simulink model "grad_V2"  (R2024a)
settings: Solver=FixedStepAuto  StartTime=0.0  StopTime=inf  RelTol=1e-3  EnableMultiTasking=on
InitFcn:
  | Ts=0.01;
  | RE=165; % count per cm
  | L=30; %cm
undefined symbols (not defined in the file or in its folder): DiscIntNeverNeededParam
libraries: arduinolib x6, arduinosensorlib x2, slpidlib x1, arduinowifilib x1
settings Model: ExtModeTrigDuration=2  Creator=andrew  LastModifiedBy=andrew
settings SolverCC: AutoInsertRateTranBlk=on
settings OptimizationCC: EnhancedBackFolding=on  PassReuseOutputArgsAs=Individual arguments  ZeroExternalMemoryAtStartup=off  ZeroInternalMemoryAtStartup=off  MaxStackSize=64  OptimizeBlockOrder=speed  DifferentSizesBufferReuse=on  OptimizationCustomize=off  EfficientTunableParamExpr=on
settings DebuggingCC: MultiTaskDSMMsg=none  ParameterTunabilityLossMsg=error
settings HardwareCC: ProdBitPerPointer=32  ProdBitPerSizeT=32  ProdBitPerPtrDiffT=32  ProdLargestAtomicInteger=Long  ProdLargestAtomicFloat=Double  ProdWordSize=32  ProdHWDeviceType=ARM Compatible->ARM Cortex
settings SFSimCC: MATLABDynamicMemAlloc=off
settings RTWCC: Description=Embedded Coder  SystemTargetFile=ert.tlc  HardwareBoard=ESP32-WROOM(Arduino Compatible)  TLCOptions="-aInlineSetEventsForThisBaseRateFcn=TLC_FALSE -aSuppressMultiTaskScheduler=TLC_FALSE  -aRateBasedStepFcn=0"  TemplateMakefile=ert_default_tmf  Toolchain=ESP32  BuildConfiguration=Faster Runs
settings CodeAppCC: ForceParamTrailComments=on  IgnoreCustomStorageClasses=off  OperatorAnnotations=on  SimulinkDataObjDesc=on  SFDataObjDesc=on  InsertBlockDesc=on
settings ERTTargetCC: SupportContinuousTime=on  SupportVariableSizeSignals=on  ExtModeTransport=3  ExtModeStaticAlloc=on  ExtModeAutomaticAllocSize=off  ExtModeStaticAllocSize=65536  ExtModeMexFile=ext_xcp  ExtModeIntrfLevel=Level2 - Open

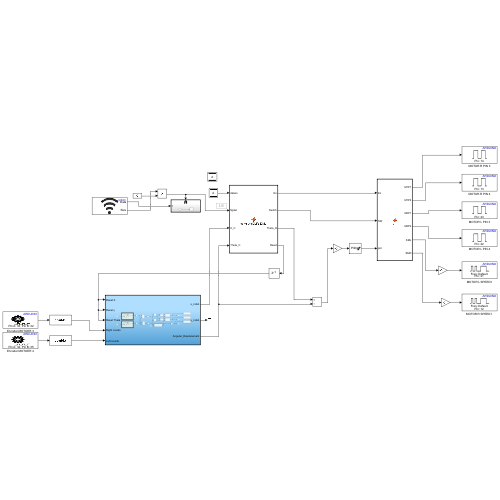
[thumbnail: Simulink's stored preview of the top-level diagram]
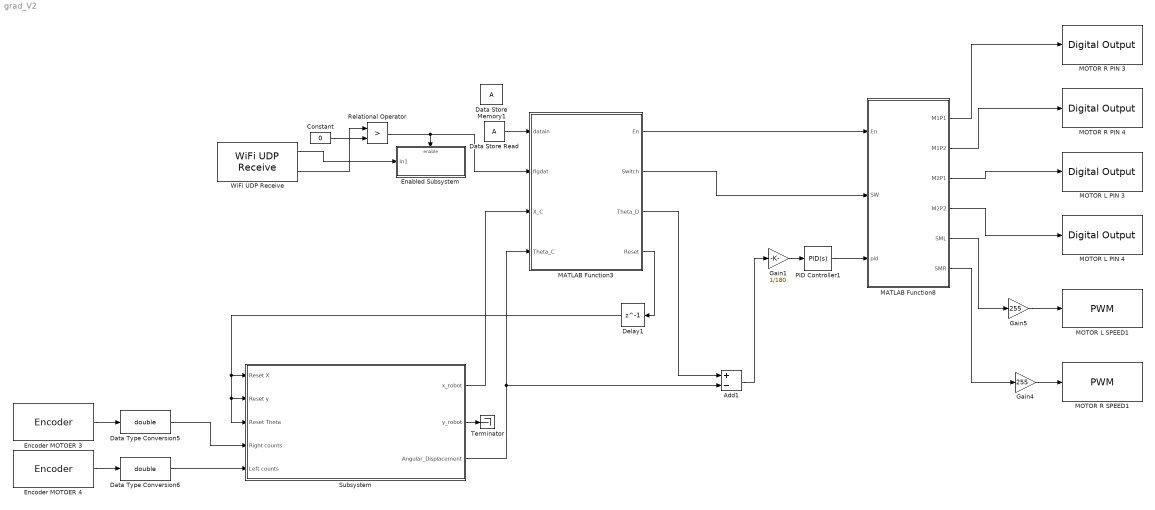
== system grad_V2 ==
  Add1 : Sum  Inputs=+-
  Constant : Constant  Value=0  OutDataTypeStr=uint16
  Data Store Memory1 : DataStoreMemory  WriteAfterWriteMsg=warning  ShowAdditionalParam=off  OutDataTypeStr=uint8  Dimensions=[20 1]
  Data Store Read : DataStoreRead  IndexOptions=Index vector (dialog)  Indices=1  OutputSizes=1
  Data Type Conversion5 : DataTypeConversion  OutDataTypeStr=double  SaturateOnIntegerOverflow=off  RndMeth=Floor
  Data Type Conversion6 : DataTypeConversion  OutDataTypeStr=double  SaturateOnIntegerOverflow=off  RndMeth=Floor
  Delay1 : Delay  DelayLength=1
  Enabled Subsystem : Subsystem  TreatAsAtomicUnit=on
  Encoder MOTOER 3 : arduinosensorlib/Encoder  InputA=33  InputB=32  Mode=No reset  SampleTime=-1
  Encoder MOTOER 4 : arduinosensorlib/Encoder  InputA=34  InputB=35  Mode=No reset  SampleTime=-1
  Gain1 : Gain  Gain=1/180
  Gain4 : Gain  Gain=255
  Gain5 : Gain  Gain=255
  MATLAB Function3 : MATLAB Function  TreatAsAtomicUnit=on
  MATLAB Function8 : MATLAB Function  TreatAsAtomicUnit=on
  MOTOR L PIN 3 : arduinolib/Digital Output  pinNumber=23  Direction=output  blockPlatform=arduino
  MOTOR L PIN 4 : arduinolib/Digital Output  pinNumber=22  Direction=output  blockPlatform=arduino
  MOTOR L SPEED1 : arduinolib/PWM  pinNumber=21  frequencyType=Default  desiredFrequency=490.2  achievableFrequency=490.2
  MOTOR R PIN 3 : arduinolib/Digital Output  pinNumber=14  Direction=output  blockPlatform=arduino
  MOTOR R PIN 4 : arduinolib/Digital Output  pinNumber=13  Direction=output  blockPlatform=arduino
  "MOTOR R SPEED1 " : arduinolib/PWM  pinNumber=12  frequencyType=Default  desiredFrequency=490.2  achievableFrequency=490.2
  PID Controller1 : slpidlib/PID Controller  Controller=PID  Form=Parallel  TimeDomain=Continuous-time  UseExternalTs=off  SampleTime=-1  IntegratorMethod=Forward Euler  FilterMethod=Forward Euler  ControllerParametersSource=internal  P=50  I=5  UseKiTs=off  D=0  UseExternalDerivativeSource=off  N=100  UseFilter=on  TunerSelectOption=Transfer Function Based (PID Tuner App)  InitialConditionSource=internal  InitialConditionForIntegrator=0  InitialConditionForFilter=0  DifferentiatorICPrevScaledInput=0  ExternalReset=none  TrackingMode=off  Kt=1  LimitOutput=on  SatLimitsSource=internal  UpperSaturationLimit=1  LowerSaturationLimit=-1  LinearizeAsGain=on  AntiWindupMode=none  Kb=1  LimitIntegrator=off  UpperIntegratorSaturationLimit=inf  LowerIntegratorSaturationLimit=-inf  POutMin=[]  POutMax=[]  IOutMin=[]  IOutMax=[]  DOutMin=[]  DOutMax=[]  NOutMin=[]  NOutMax=[]  SumOutMin=[]  SumOutMax=[]  SaturationOutMin=[]  SaturationOutMax=[]  PParamMin=[]  PParamMax=[]  IParamMin=[]  IParamMax=[]  DParamMin=[]  DParamMax=[]  NParamMin=[]  NParamMax=[]  KbParamMin=[]  KbParamMax=[]  KtParamMin=[]  KtParamMax=[]  KbOutMin=[]  KbOutMax=[]  KtOutMin=[]  KtOutMax=[]  IntegratorOutMin=[]  IntegratorOutMax=[]  FilterOutMin=[]  FilterOutMax=[]  SumI1OutMin=[]  SumI1OutMax=[]  SumI2OutMin=[]  SumI2OutMax=[]  SumI3OutMin=[]  SumI3OutMax=[]  SumI4OutMin=[]  SumI4OutMax=[]  SumDOutMin=[]  SumDOutMax=[]  DifferentiatorOutMin=[]  DifferentiatorOutMax=[]  FilterDiffOutCoefMin=[]  FilterDiffOutCoefMax=[]  ReciprocalOutMin=[]  ReciprocalOutMax=[]  SumDenOutMin=[]  SumDenOutMax=[]  SumNumOutMin=[]  SumNumOutMax=[]  DivideOutMin=[]  DivideOutMax=[]  UdiffTsProdOutMin=[]  UdiffTsProdOutMax=[]  NTsProdOutMin=[]  NTsProdOutMax=[]  UintegralTsProdOutMin=[]  UintegralTsProdOutMax=[]  UngainTsProdOutMin=[]  UngainTsProdOutMax=[]  ClampingZeroOutDataTypeStr=Inherit: Inherit via back propagation  ClampingZeroOutMin=[]  ClampingZeroOutMax=[]  FilterDenConstantOutDataTypeStr=Inherit: Inherit via back propagation  FilterDenConstantOutMin=[]  FilterDenConstantOutMax=[]  PCopyOutDataTypeStr=Inherit: Inherit via back propagation  PCopyOutMin=[]  PCopyOutMax=[]  NCopyOutDataTypeStr=Inherit: Inherit via back propagation  NCopyOutMin=[]  NCopyOutMax=[]  IntegratorContinuousStateAttributes=''  IntegratorStateMustResolveToSignalObject=off  IntegratorRTWStateStorageClass=Auto  FilterContinuousStateAttributes=''  FilterStateMustResolveToSignalObject=off  FilterRTWStateStorageClass=Auto  ParallelPVariant=InternalParameters  IdealPVariant=Disabled  IVariant=InternalParameters  DVariant=InternalParameters  IntegratorVariant=Continuous  SatVariant=Enabled  AWVariant=Passthrough  PCopyVariant=Disabled  TRVariant=Disabled  FdbkBlocksVariant=Forward  IdealPFdbkVariant=Disabled  SatFdbkVariant=Disabled  DerivativeFilterVariant=ContFilter  NVariant=InternalParameters  NCopyVariant=Disabled  FilterICVariant=InternalICsFilter  IntegratorICVariant=InternalICs  ExternalResetVariant=Disabled  TRSumVariant=Passthrough  SumFdbkVariant=Disabled  SumVariant=Sum_PID  TsampFilterVariant=InternalTs  TsampNgainVariant=Passthrough  TsampIntegralVariant=Disabled_SignalSpec  ExternalSaturationOutDataTypeStr=Inherit: Same as second input  DerivativeSourceVariant=ErrorSignal
  Relational Operator : RelationalOperator  Operator=>  OutDataTypeStr=boolean  RndMeth=Simplest  InputSameDT=off
  Subsystem : Subsystem  TreatAsAtomicUnit=on  SystemSampleTime=Ts
  Terminator : Terminator
  WiFi UDP Receive : arduinowifilib/WiFi UDP Receive  localport=50002  DataType=uint8  DataLength=20  SampleTime_=0.1  wifiUDPIndex=0  blockPlatform=ARDUINO  isARMArch=false
  wires:
  Subsystem/3(Angular_Displacement) -> MATLAB Function3/4(Theta_C), Add1/2
  WiFi UDP Receive/1 -> Enabled Subsystem/1(In1)
  MATLAB Function8/4(M2P2) -> MOTOR L PIN 4/1
  MATLAB Function3/4(Reset) -> Delay1/1
  Constant/1 -> Relational Operator/2
  WiFi UDP Receive/2 -> Relational Operator/1
  MATLAB Function8/3(M2P1) -> MOTOR L PIN 3/1
  MATLAB Function8/6(SMR) -> Gain4/1
  Data Store Read/1 -> MATLAB Function3/1(datain)
  MATLAB Function8/1(M1P1) -> MOTOR R PIN 3/1
  Encoder MOTOER 3/1 -> Data Type Conversion5/1
  Gain5/1 -> MOTOR L SPEED1/1
  Relational Operator/1 -> MATLAB Function3/2(flgdat), Enabled Subsystem/Enable
  MATLAB Function8/5(SML) -> Gain5/1
  Encoder MOTOER 4/1 -> Data Type Conversion6/1
  MATLAB Function3/2(Switch) -> MATLAB Function8/2(SW)
  Add1/1 -> Gain1/1
  MATLAB Function3/1(En) -> MATLAB Function8/1(En)
  Subsystem/2(y_robot) -> Terminator/1
  Data Type Conversion5/1 -> Subsystem/4(Right counts)
  Delay1/1 -> Subsystem/3(Reset Theta), Subsystem/2(Reset y), Subsystem/1(Reset X)
  Gain4/1 -> "MOTOR R SPEED1 "/1
  Subsystem/1(x_robot) -> MATLAB Function3/3(X_C)
  Gain1/1 -> PID Controller1/1
  MATLAB Function8/2(M1P2) -> MOTOR R PIN 4/1
  MATLAB Function3/3(Theta_D) -> Add1/1
  PID Controller1/1 -> MATLAB Function8/3(pid)
  Data Type Conversion6/1 -> Subsystem/5(Left counts)

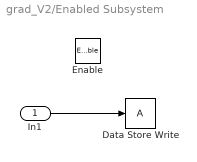
== system grad_V2/Enabled Subsystem ==
  In1 : Inport
  Enable : EnablePort
  Data Store Write : DataStoreWrite  IndexOptions=Index vector (dialog)  Indices=1  OutputSizes=1
  wires:
  In1/1 -> Data Store Write/1

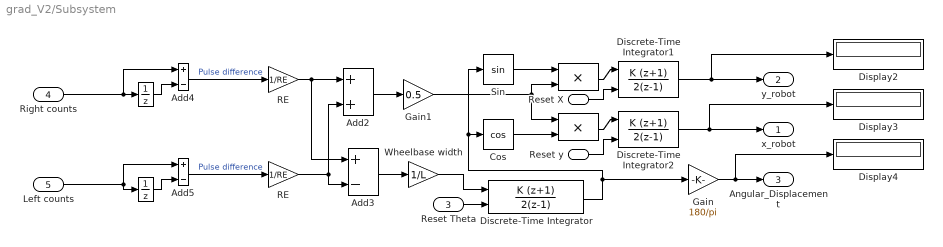
== system grad_V2/Subsystem ==
  Reset X : Inport
  Reset y : Inport  Port=2
  Reset Theta : Inport  Port=3
  Right counts : Inport  Port=4
  Left counts : Inport  Port=5
  " " : Product
  "  " : Product
  "     " : UnitDelay  SampleTime=-1  HasFrameUpgradeWarning=on
  "       " : UnitDelay  SampleTime=-1  HasFrameUpgradeWarning=on
  Add2 : Sum
  Add3 : Sum  Inputs=+-
  Add4 : Sum  Inputs=+-
  Add5 : Sum  Inputs=+-
  Cos : Trigonometry  Operator=cos  ApproximationMethod=CORDIC
  Discrete-Time Integrator : DiscreteIntegrator  IntegratorMethod=Accumulation: Trapezoidal  ExternalReset=level  SampleTime=-1  ICPrevOutput=DiscIntNeverNeededParam  ICPrevScaledInput=DiscIntNeverNeededParam
  Discrete-Time Integrator1 : DiscreteIntegrator  IntegratorMethod=Accumulation: Trapezoidal  ExternalReset=level  SampleTime=-1  ICPrevOutput=DiscIntNeverNeededParam  ICPrevScaledInput=DiscIntNeverNeededParam
  Discrete-Time Integrator2 : DiscreteIntegrator  IntegratorMethod=Accumulation: Trapezoidal  ExternalReset=level  SampleTime=-1  ICPrevOutput=DiscIntNeverNeededParam  ICPrevScaledInput=DiscIntNeverNeededParam
  Display2 : Display
  Display3 : Display
  Display4 : Display
  Gain : Gain  Gain=180/pi
  Gain1 : Gain  Gain=0.5
  "RE  " : Gain  Gain=1/RE
  "RE    " : Gain  Gain=1/RE
  Sin : Trigonometry  ApproximationMethod=CORDIC
  "Wheelbase width " : Gain  Gain=1/L
  x_robot : Outport  VectorParamsAs1DForOutWhenUnconnected=off
  y_robot : Outport  Port=2  VectorParamsAs1DForOutWhenUnconnected=off
  Angular_Displacement : Outport  Port=3  VectorParamsAs1DForOutWhenUnconnected=off
  wires:
  " "/1 -> Discrete-Time Integrator2/1
  Gain1/1 -> " "/1, "  "/2
  "  "/1 -> Discrete-Time Integrator1/1
  Right counts/1 -> Add4/1, "     "/1
  "RE    "/1 -> Add3/2, Add2/2
  Discrete-Time Integrator/1 -> Gain/1, Sin/1, Cos/1
  Add2/1 -> Gain1/1
  Cos/1 -> " "/2
  "Wheelbase width "/1 -> Discrete-Time Integrator/1
  "RE  "/1 -> Add2/1, Add3/1
  Discrete-Time Integrator1/1 -> y_robot/1, Display2/1
  "       "/1 -> Add5/2
  Discrete-Time Integrator2/1 -> x_robot/1, Display3/1
  Left counts/1 -> "       "/1, Add5/1
  Add5/1 -> "RE    "/1  "Pulse difference"
  "     "/1 -> Add4/2
  Sin/1 -> "  "/1
  Add3/1 -> "Wheelbase width "/1
  Add4/1 -> "RE  "/1  "Pulse difference"
  Gain/1 -> Display4/1, Angular_Displacement/1
  Reset Theta/1 -> Discrete-Time Integrator/2
  Reset y/1 -> Discrete-Time Integrator2/2
  Reset X/1 -> Discrete-Time Integrator1/2

== matlab function grad_V2/MATLAB Function3 ==
  settings: updateMethod=DISCRETE
  data: En output size=1; Switch output size=1; Theta_D output size=1; Reset output size=1; datain input; flgdat input; X_C input; Theta_C input
function [En,Switch,Theta_D,Reset] = computeDMR_DML(datain,flgdat,X_C,Theta_C)
    % MATLAB Function block: compute DMR, DML, Theta_D with persistent state
    persistent i n flag_D flag_Th flag_SW XD ThetaD data flag_fin 
    % Initialize persistent variables if they are empty
    if isempty(i)
        i = 1;
        flag_D = 0;
        flag_Th = 0;
        flag_SW = 0;
        flag_fin = 1;
        n=20;
        XD = int8(0);
        ThetaD = int8(0);
        Reset = 1;
        data = int8(zeros(1,20));        
    end
    if (flgdat && flag_fin)
        data = typecast(datain,'int8');
        i=1;
        XD = data(i);
        ThetaD = data(i+1);
        flag_fin = 0;
        if (XD == 0)
            flag_SW = 1;
        else 
            flag_SW = 0;
        end
    end
    data_out = int8(zeros(1,20));
    En = 0;
    Reset = 0;
    
    % **Ensure output variables are initialized to default values**
    

    % Compare X_C with X_D
    if abs(XD-X_C) <= 2
        flag_D = 1;
    else 
        flag_D = 0;
    end
    
    % Compare Theta_C with Theta_D
    if abs(ThetaD-Theta_C) <= 1 
        flag_Th = 1;
    else 
        flag_Th = 0;
    end
   
    if (flag_Th == 0 || flag_D == 0) 
        En = 1;
    end

    if (i<n-2 && (flag_Th == 1 && flag_SW==1) || (flag_D == 1 && flag_SW==0))
        i=i+2;
        % Retrieve current reference values from data array
        XD = data(i);
        if (XD == 0)
            flag_SW = 1;
        else 
            flag_SW = 0;
        end
        ThetaD = data(i+1);
        Reset = 1;
    elseif (i>=n-2 && (flag_Th == 1 && flag_SW==1) || (flag_D == 1 && flag_SW==0))
        En = 0;
        Reset = 1;
        flag_fin = 1;
    end
    Switch = flag_SW;
    Theta_D=ThetaD;
    flgD=flag_D;
    flgth=flag_Th;
    data_out = data(1:20);
    idx = i;
  end

== matlab function grad_V2/MATLAB Function8 ==
  data: En input; M1P1 output; M1P2 output; M2P1 output; M2P2 output; SW input; pid input; SML output; SMR output
function [M1P1 , M1P2,M2P1,M2P2,SML,SMR] = fcn(En,SW,pid)
    BUZZER = 0;
  if (SW == 0)
    vn=1-abs(pid); 
  else
    vn=0;    
  end
  vr=vn+pid;
  vl=vn-pid; 

  if (vr>=0)
     % Forward
    M1P1 = 1; M1P2 = 0;
  else
      % Backward
    M1P1 = 0; M1P2 = 1;
  end
  
  if (vl>=0)
      % Forward
    M2P1 = 1; M2P2 = 0;
  else
      % Backward
    M2P1 = 0; M2P2 = 1;
  end

  % if (US <= 10)
  %      M1P1 = 1; M1P2 = 1;
  %      M2P1 = 1; M2P2 = 1;
  %      BUZZER = 200;
  % end
  SML = abs(vl)*En;
  SMR = abs(vr)*En;
end
